simulink model "SimulacionesDT_LUCIA_con_integral"  (R2026b)
settings: Solver=ode15s  StopTime=20
values from neighbouring files (symbols this model uses):
  alpha_Cu = 3.9e-3    (= 0.0039)    [coeficientes.m]
  b_eq = b_m + b_l/(r^2)    (= 2.19444444444e-05)    [coeficientes.m]
  C_ts = 0.818    [coeficientes.m]
  g = 9.80665    [coeficientes.m]
  init_I0 = 0    [coeficientes.m]
  init_Id = 0    [coeficientes.m]
  init_Iq = 0    [coeficientes.m]
  init_theta = 0    [coeficientes.m]
  init_Ts = 20    [coeficientes.m]
  init_w = 0    [coeficientes.m]
  J_eq = J_m + J_l/(r^2)    (= 2.84652777778e-05)    [coeficientes.m]
  k_l = k_l_min + m_l*l_l    (= 0.5)    [coeficientes.m]
  Kd_mov = wn_mov * (2*zeta_mov + 1) * J_eq    (= 0.0569305555556)    [coeficientes.m]
  Ki_mov = wn_mov^3 * J_eq    (= 14574.2222222)    [coeficientes.m]
  Kp_mov = wn_mov^2 * (2*zeta_mov + 1) * J_eq    (= 45.5444444444)    [coeficientes.m]
  L_d = 6.6e-3    (= 0.0066)    [coeficientes.m]
  L_ls = 0.8e-3    (= 0.0008)    [coeficientes.m]
  L_q = 5.8e-3    (= 0.0058)    [coeficientes.m]
  lambda = 0.016    [coeficientes.m]
  Pp = 3    [coeficientes.m]
  r = 120.0    (= 120)    [coeficientes.m]
  R0 = abs(p)*L_ls    [coeficientes.m]
  R_sREF = 1.02    [coeficientes.m]
  R_tsamb = 146.7    [coeficientes.m]
  Rd = abs(p)*L_d    [coeficientes.m]
  Rq = abs(p)*L_q    [coeficientes.m]
  T_sREF = 20    [coeficientes.m]
libraries: eeTransforms x12
(part 1 of 2)
settings Model: Creator=lamun  LastModifiedBy=lamun
settings SimscapeCC: SimscapeLogType=all  SimscapeNominalValues="[{\"value\":\"1\",\"unit\":\"A\"},{\"value\":\"1\",\"unit\":\"bar\"},{\"value\":\"1\",\"unit\":\"cm^2\"},{\"value\":\"1\",\"unit\":\"cm^3/s\"},{\"value\":\"1\",\"unit\":\"kJ/kg\"},{\"value\":\"1\",\"unit\":\"kW\"},{\"value\":\"1\",\"unit\":\"l\"},{\"value\":\"1\",\"unit\":\"N\"},{\"value\":\"1\",\"unit\":\"N*m\"},{\"value\":\"1\",\"unit\":\"V\"},{\"value\":\"0.001\",\"unit\":\"Wb\"}]"  SimscapeUseEnergyAccounting=off

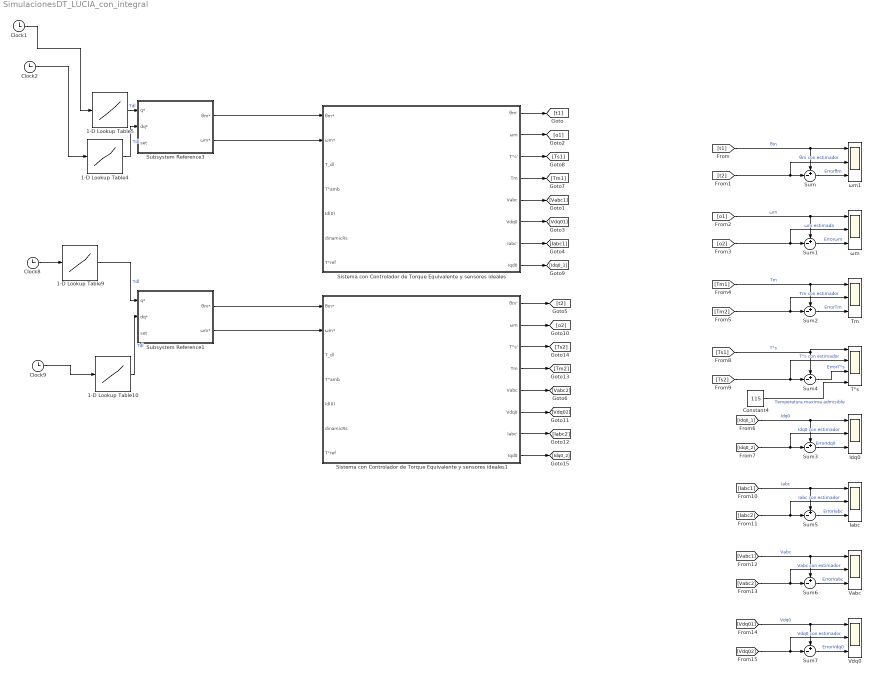
== system SimulacionesDT_LUCIA_con_integral ==
  1-D Lookup Table10 : Lookup_n-D  NumberOfTableDimensions=1  BreakpointsForDimension1=[0, 1.99, 2, 6.99, 7, 8.99, 9, 13.99, 14, 16]  Table=[0, 0, 2*pi/5, 2*pi/5, 0, 0, -2*pi/5, -2*pi/5, 0, 0]  InternalRulePriority=Speed  RndMeth=Simplest
  1-D Lookup Table4 : Lookup_n-D  NumberOfTableDimensions=1  BreakpointsForDimension1=[0, 1.99, 2, 6.99, 7, 8.99, 9, 13.99, 14, 16]  Table=[0, 0, 2*pi/5, 2*pi/5, 0, 0, -2*pi/5, -2*pi/5, 0, 0]  InternalRulePriority=Speed  RndMeth=Simplest
  1-D Lookup Table5 : Lookup_n-D  NumberOfTableDimensions=1  BreakpointsForDimension1=[0, 2, 7, 9, 14, 16]  Table=[0, 0, 2*pi, 2*pi, 0, 0]  InternalRulePriority=Speed  RndMeth=Simplest
  1-D Lookup Table9 : Lookup_n-D  NumberOfTableDimensions=1  BreakpointsForDimension1=[0, 2, 7, 9, 14, 16]  Table=[0, 0, 2*pi, 2*pi, 0, 0]  InternalRulePriority=Speed  RndMeth=Simplest
  Clock{1..2,8..9} (4 alike) : Clock
  Constant4 : Constant  Value=115
  Iabc : Scope  NumInputPorts=3
      settings: Title=Comparación Iabc  ActiveDisplayYMinimum=-616.4753395036073  ActiveDisplayYMaximum=771.0246685119215  YLabel=Iabc [A]  DataLoggingVariableName=ScopeData6
  Idq0 : Scope  NumInputPorts=3
      settings: Title=Comparación Idq0  ActiveDisplayYMinimum=-302.22808719672526  ActiveDisplayYMaximum=701.5039994194284  YLabel=Idq0 [A]  DataLoggingVariableName=ScopeData3
  Sistema con Controlador de Torque Equivalente y sensores ideales : Subsystem
  Sistema con Controlador de Torque Equivalente y sensores ideales1 : Subsystem
  Subsystem Reference1 : Subsystem
  Subsystem Reference3 : Subsystem
  Sum{,1..7} (8 alike) : Sum  Inputs=+-|
  Tm : Scope  NumInputPorts=3
      settings: Title=Comparación Torque Motor  ActiveDisplayYMinimum=-3.6327134054434631  ActiveDisplayYMaximum=3.6460056409791535  YLabel=T_m [Nm]
  T°s : Scope  NumInputPorts=4
      settings: Title=Comparación Temperatura del Estator  ActiveDisplayYMinimum=-1.4333497629401416E+11  ActiveDisplayYMaximum=1.2900147868458242E+12  YLabel=T\circ  DataLoggingVariableName=ScopeData2
  Vabc : Scope  NumInputPorts=3
      settings: Title=Comparación Vabc  ActiveDisplayYMinimum=-4.2380725007516653E+17  ActiveDisplayYMaximum=4.48793359005676E+17  YLabel=Vabc [V]  DataLoggingVariableName=ScopeData7
  Vdq0 : Scope  NumInputPorts=3
      settings: Title=Comparación Vdq0  ActiveDisplayYMinimum=-9.3011147894303968E+16  ActiveDisplayYMaximum=4.5901314557328838E+17  YLabel=Vdq0 [V]  DataLoggingVariableName=ScopeData8
  ωm : Scope  NumInputPorts=3
      settings: Title=Comparación ωm  ActiveDisplayYMinimum=-384.34516117127549  ActiveDisplayYMaximum=399.454060833598  YLabel=\omega_{motor}  DataLoggingVariableName=ScopeData5
  ωm1 : Scope  NumInputPorts=3
      settings: Title=Comparación θ motor  ActiveDisplayYMinimum=-120.08554135265514  ActiveDisplayYMaximum=869.13028937421041  YLabel=\theta_m[rad]  DataLoggingVariableName=ScopeData4
  wires:
  Sistema con Controlador de Torque Equivalente y sensores ideales1/7(Iabc') -> [Iabc2]
  [Vabc1] -> Sum6/1, Vabc/1  "Vabc"
  Sistema con Controlador de Torque Equivalente y sensores ideales1/6(Vdq0) -> [Vdq02]
  Sistema con Controlador de Torque Equivalente y sensores ideales/7(Iabc') -> [Iabc1]
  Sum1/1 -> ωm/3  "Errorωm"
  Sistema con Controlador de Torque Equivalente y sensores ideales1/8(Iqd0) -> [Idq0_2]
  Sum/1 -> ωm1/3  "Errorθm"
  Sistema con Controlador de Torque Equivalente y sensores ideales/6(Vdq0) -> [Vdq01]
  [Iabc1] -> Sum5/1, Iabc/1  "Iabc"
  Sum5/1 -> Iabc/3  "ErrorIabc"
  [Tm1] -> Tm/1, Sum2/1  "Tm"
  Subsystem Reference3/1(θm*) -> Sistema con Controlador de Torque Equivalente y sensores ideales/1(θm*)
  Sistema con Controlador de Torque Equivalente y sensores ideales/8(Iqd0) -> [Idq0_1]
  [Idq0_2] -> Idq0/2, Sum3/2  "Idq0 con estimador"
  Sum6/1 -> Vabc/3  "ErrorVabc"
  [Idq0_1] -> Sum3/1, Idq0/1  "Idq0"
  Sistema con Controlador de Torque Equivalente y sensores ideales1/3(T°s') -> [Ts2]
  [o1] -> ωm/1, Sum1/1  "ωm"
  [Vdq02] -> Vdq0/2, Sum7/2  "Vdq0 con estimador"
  Sistema con Controlador de Torque Equivalente y sensores ideales/5(Vabc) -> [Vabc1]
  Sistema con Controlador de Torque Equivalente y sensores ideales/3(T°s') -> [Ts1]
  Sistema con Controlador de Torque Equivalente y sensores ideales/1(θm') -> [t1]
  Sistema con Controlador de Torque Equivalente y sensores ideales1/2(ωm) -> [o2]
  [Tm2] -> Tm/2, Sum2/2  "Tm con estimador"
  Subsystem Reference3/2(ωm*) -> Sistema con Controlador de Torque Equivalente y sensores ideales/2(ωm*)
  Subsystem Reference1/1(θm*) -> Sistema con Controlador de Torque Equivalente y sensores ideales1/1(θm*)
  [Vdq01] -> Sum7/1, Vdq0/1  "Vdq0"
  [t2] -> ωm1/2, Sum/2  "θm con estimador"
  [t1] -> ωm1/1, Sum/1  "θm"
  Sum7/1 -> Vdq0/3  "ErrorVdq0"
  Sistema con Controlador de Torque Equivalente y sensores ideales1/4(Tm) -> [Tm2]
  Sum3/1 -> Idq0/3  "ErrorIdq0"
  Sum2/1 -> Tm/3  "ErrorTm"
  [Ts2] -> T°s/2, Sum4/2  "T°s con estimador"
  [o2] -> ωm/2, Sum1/2  "ωm estimada"
  Sum4/1 -> T°s/3  "ErrorT°s"
  Sistema con Controlador de Torque Equivalente y sensores ideales1/1(θm') -> [t2]
  Sistema con Controlador de Torque Equivalente y sensores ideales1/5(Vabc) -> [Vabc2]
  [Ts1] -> T°s/1, Sum4/1  "T°s"
  Sistema con Controlador de Torque Equivalente y sensores ideales/2(ωm) -> [o1]
  Subsystem Reference1/2(ωm*) -> Sistema con Controlador de Torque Equivalente y sensores ideales1/2(ωm*)
  [Iabc2] -> Iabc/2, Sum5/2  "Iabc con estimador"
  Sistema con Controlador de Torque Equivalente y sensores ideales/4(Tm) -> [Tm1]
  [Vabc2] -> Vabc/2, Sum6/2  "Vabc con estimador"
  Constant4/1 -> T°s/4  "Temperatura maxima admisible"
  Clock2/1 -> 1-D Lookup Table4/1
  Clock1/1 -> 1-D Lookup Table5/1
  Clock9/1 -> 1-D Lookup Table10/1
  Clock8/1 -> 1-D Lookup Table9/1
  1-D Lookup Table9/1 -> Subsystem Reference1/1(q*)  "Tdl"
  1-D Lookup Table10/1 -> Subsystem Reference1/2(dq*)  "Tdl"
  1-D Lookup Table4/1 -> Subsystem Reference3/2(dq*)  "Tdl"
  1-D Lookup Table5/1 -> Subsystem Reference3/1(q*)  "Tdl"

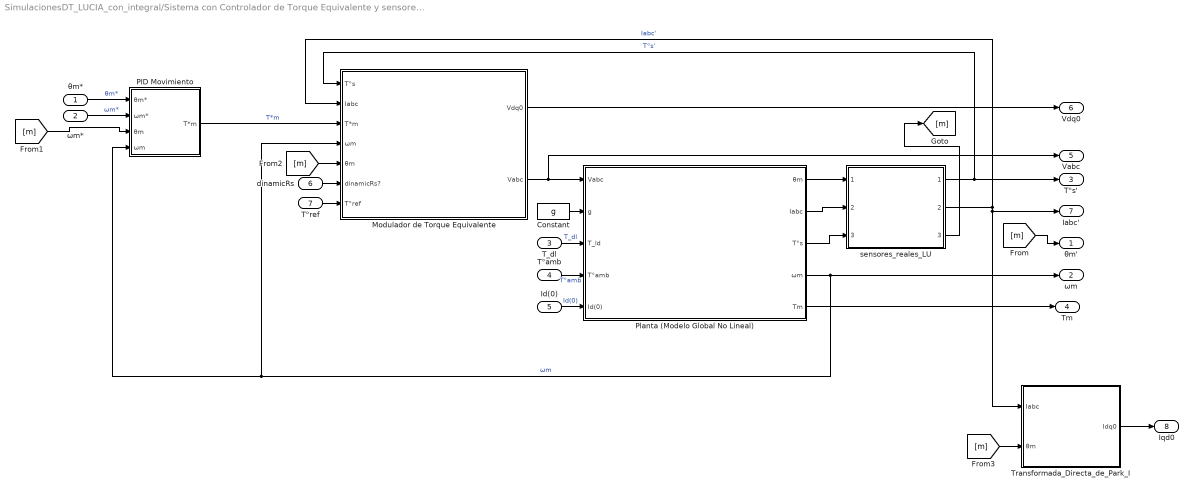
== system SimulacionesDT_LUCIA_con_integral/Sistema con Controlador de Torque Equivalente y sensores ideales ==
  θm* : Inport
  ωm* : Inport  Port=2
  T_dl : Inport  Port=3
  T°amb : Inport  Port=4
  Id(0) : Inport  Port=5
  dinamicRs : Inport  Port=6
  T°ref : Inport  Port=7
  Constant : Constant  Value=g
  Modulador de Torque Equivalente : Subsystem
      settings: PortSchema="{\"entries\":[{\"content\":{\"sides\":[{\"content\":{\"connectorIds\":[\"In1\",\"In3\",\"In5\",\"In2\",\"In4\",\"In6\",\"In7\"]},\"type\":\"ConnectorPlacement.EquallySpacedRectSide\",\"uuid\":\"ea9ad4ab-f607-4d37-9442-85f6cfda2486\"},{\"content\":{\"connectorIds\":[\"Out2\",\"Out1\"],\"side\":\"RIGHT\"},\"type\":\"ConnectorPlacement.EquallySpacedRectSide\",\"uuid\":\"696b5fe5-1f6c-4fc9-932e-86b56d49996f\"},{\"content\":{\"side\":\"TOP\"},\"type\":\"ConnectorPlacement.EquallySpacedRectSide\",\"uuid\":\"45e3ac4c-5a2f-4a79-9454-e497b07295c7\"}]},\"type\":\"ConnectorPlacement.EquallySpacedConnector\",\"uuid\":\"ad401c21-3c60-4ab4-96eb-f449fc93609a\"}],\"packageUris\":[\"http://schema.mathworks.com/mf0/Connector/R2020b\"],\"version\":\"1.0\"}"
  PID Movimiento : Subsystem
      settings: PortSchema="{\"entries\":[{\"content\":{\"sides\":[{\"content\":{\"connectorIds\":[\"In3\",\"In4\",\"In2\",\"In1\"]},\"type\":\"ConnectorPlacement.EquallySpacedRectSide\",\"uuid\":\"99b9ec4b-f651-40ed-8a16-085c2c4ac88d\"},{\"content\":{\"connectorIds\":[\"Out1\"],\"side\":\"RIGHT\"},\"type\":\"ConnectorPlacement.EquallySpacedRectSide\",\"uuid\":\"009a9369-fd86-4ac2-a423-7c7f1491457b\"},{\"content\":{\"side\":\"TOP\"},\"type\":\"ConnectorPlacement.EquallySpacedRectSide\",\"uuid\":\"0bc889a5-9100-482e-a11a-4c36993d76f7\"}]},\"type\":\"ConnectorPlacement.EquallySpacedConnector\",\"uuid\":\"de270b8a-8a15-46e7-87f3-10db7988a399\"}],\"packageUris\":[\"http://schema.mathworks.com/mf0/Connector/R2020b\"],\"version\":\"1.0\"}"
  Planta (Modelo Global No Lineal) : Subsystem
      settings: PortSchema="{\"entries\":[{\"content\":{\"sides\":[{\"content\":{\"connectorIds\":[\"In1\",\"In3\",\"In2\",\"In4\",\"In5\"]},\"type\":\"ConnectorPlacement.EquallySpacedRectSide\",\"uuid\":\"3481abf0-b0cb-49f6-b93f-5a31fbfa4119\"},{\"content\":{\"connectorIds\":[\"Out1\",\"Out2\",\"Out3\",\"Out4\",\"Out5\"],\"side\":\"RIGHT\"},\"type\":\"ConnectorPlacement.EquallySpacedRectSide\",\"uuid\":\"81dbc61e-d5f3-4edc-bc73-ec3d6160a008\"},{\"content\":{\"side\":\"TOP\"},\"type\":\"ConnectorPlacement.EquallySpacedRectSide\",\"uuid\":\"48e37594-92fb-4835-b4aa-9211b8b6a309\"}]},\"type\":\"ConnectorPlacement.EquallySpacedConnector\",\"uuid\":\"6c32b8e1-5803-41f4-af4e-ba3a494349ba\"}],\"packageUris\":[\"http://schema.mathworks.com/mf0/Connector/R2020b\"],\"version\":\"1.0\"}"
  Transformada_Directa_de_Park_I : Subsystem
  sensores_reales_LU : Subsystem  ReferencedSubsystem=sensores_reales_LU
  θm' : Outport
  ωm : Outport  Port=2
  T°s' : Outport  Port=3
  Tm : Outport  Port=4
  Vabc : Outport  Port=5  OutDataTypeStr=Bus: Vabc
  Vdq0 : Outport  Port=6  OutDataTypeStr=Bus: Vdq0
  Iabc' : Outport  Port=7  OutDataTypeStr=Bus: Iabc
  Iqd0 : Outport  Port=8  OutDataTypeStr=Bus: Idq0
  wires:
  Transformada_Directa_de_Park_I/1(Idq0) -> Iqd0/1
  T°ref/1 -> Modulador de Torque Equivalente/7(T°ref)
  dinamicRs/1 -> Modulador de Torque Equivalente/6(dinamicRs?)
  Modulador de Torque Equivalente/2(Vdq0) -> Vdq0/1
  Planta (Modelo Global No Lineal)/5(Tm) -> Tm/1
  T_dl/1 -> Planta (Modelo Global No Lineal)/2(T_ld)  "T_dl"
  T°amb/1 -> Planta (Modelo Global No Lineal)/4(T°amb)  "T°amb"
  Id(0)/1 -> Planta (Modelo Global No Lineal)/5(Id(0))  "Id(0)"
  Constant/1 -> Planta (Modelo Global No Lineal)/3(g)
  sensores_reales_LU/1 -> T°s'/1, Modulador de Torque Equivalente/1(T°s)  "T°s'"
  sensores_reales_LU/2 -> Transformada_Directa_de_Park_I/1(Iabc), Iabc'/1, Modulador de Torque Equivalente/3(Iabc)  "Iabc'"
  Planta (Modelo Global No Lineal)/3(T°s) -> sensores_reales_LU/3
  Modulador de Torque Equivalente/1(Vabc) -> Vabc/1, Planta (Modelo Global No Lineal)/1(Vabc)
  Planta (Modelo Global No Lineal)/2(Iabc) -> sensores_reales_LU/2
  Planta (Modelo Global No Lineal)/1(θm) -> sensores_reales_LU/1
  θm*/1 -> PID Movimiento/3(θm*)  "θm*"
  PID Movimiento/1(T*m) -> Modulador de Torque Equivalente/5(T*m)  "T*m"
  ωm*/1 -> PID Movimiento/4(ωm*)  "ωm*"
  Planta (Modelo Global No Lineal)/4(ωm) -> PID Movimiento/1(ωm), Modulador de Torque Equivalente/2(ωm), ωm/1  "ωm"
  sensores_reales_LU/3 -> [m]
  [m] -> θm'/1
  [m] -> PID Movimiento/2(θm)
  [m] -> Modulador de Torque Equivalente/4(θm)
  [m] -> Transformada_Directa_de_Park_I/2(θm)

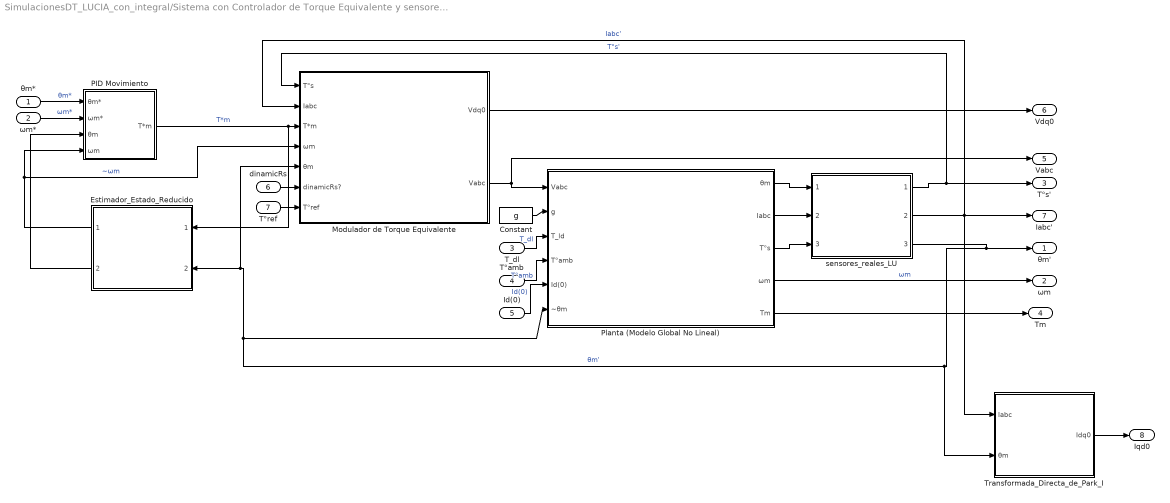
== system SimulacionesDT_LUCIA_con_integral/Sistema con Controlador de Torque Equivalente y sensores ideales1 ==
  θm* : Inport
  ωm* : Inport  Port=2
  T_dl : Inport  Port=3
  T°amb : Inport  Port=4
  Id(0) : Inport  Port=5
  dinamicRs : Inport  Port=6
  T°ref : Inport  Port=7
  Constant : Constant  Value=g
  Estimador_Estado_Reducido : Subsystem  ReferencedSubsystem=Estimador_Estado_Reducido
  Modulador de Torque Equivalente : Subsystem
      settings: PortSchema="{\"entries\":[{\"content\":{\"sides\":[{\"content\":{\"connectorIds\":[\"In1\",\"In3\",\"In5\",\"In2\",\"In4\",\"In6\",\"In7\"]},\"type\":\"ConnectorPlacement.EquallySpacedRectSide\",\"uuid\":\"ea9ad4ab-f607-4d37-9442-85f6cfda2486\"},{\"content\":{\"connectorIds\":[\"Out2\",\"Out1\"],\"side\":\"RIGHT\"},\"type\":\"ConnectorPlacement.EquallySpacedRectSide\",\"uuid\":\"696b5fe5-1f6c-4fc9-932e-86b56d49996f\"},{\"content\":{\"side\":\"TOP\"},\"type\":\"ConnectorPlacement.EquallySpacedRectSide\",\"uuid\":\"45e3ac4c-5a2f-4a79-9454-e497b07295c7\"}]},\"type\":\"ConnectorPlacement.EquallySpacedConnector\",\"uuid\":\"ad401c21-3c60-4ab4-96eb-f449fc93609a\"}],\"packageUris\":[\"http://schema.mathworks.com/mf0/Connector/R2020b\"],\"version\":\"1.0\"}"
  PID Movimiento : Subsystem
      settings: PortSchema="{\"entries\":[{\"content\":{\"sides\":[{\"content\":{\"connectorIds\":[\"In3\",\"In4\",\"In2\",\"In1\"]},\"type\":\"ConnectorPlacement.EquallySpacedRectSide\",\"uuid\":\"99b9ec4b-f651-40ed-8a16-085c2c4ac88d\"},{\"content\":{\"connectorIds\":[\"Out1\"],\"side\":\"RIGHT\"},\"type\":\"ConnectorPlacement.EquallySpacedRectSide\",\"uuid\":\"009a9369-fd86-4ac2-a423-7c7f1491457b\"},{\"content\":{\"side\":\"TOP\"},\"type\":\"ConnectorPlacement.EquallySpacedRectSide\",\"uuid\":\"0bc889a5-9100-482e-a11a-4c36993d76f7\"}]},\"type\":\"ConnectorPlacement.EquallySpacedConnector\",\"uuid\":\"de270b8a-8a15-46e7-87f3-10db7988a399\"}],\"packageUris\":[\"http://schema.mathworks.com/mf0/Connector/R2020b\"],\"version\":\"1.0\"}"
  Planta (Modelo Global No Lineal) : Subsystem
      settings: PortSchema="{\"entries\":[{\"content\":{\"sides\":[{\"content\":{\"connectorIds\":[\"In1\",\"In3\",\"In2\",\"In4\",\"In5\",\"In6\"]},\"type\":\"ConnectorPlacement.EquallySpacedRectSide\",\"uuid\":\"3481abf0-b0cb-49f6-b93f-5a31fbfa4119\"},{\"content\":{\"connectorIds\":[\"Out1\",\"Out2\",\"Out3\",\"Out4\",\"Out5\"],\"side\":\"RIGHT\"},\"type\":\"ConnectorPlacement.EquallySpacedRectSide\",\"uuid\":\"81dbc61e-d5f3-4edc-bc73-ec3d6160a008\"},{\"content\":{\"side\":\"TOP\"},\"type\":\"ConnectorPlacement.EquallySpacedRectSide\",\"uuid\":\"48e37594-92fb-4835-b4aa-9211b8b6a309\"}]},\"type\":\"ConnectorPlacement.EquallySpacedConnector\",\"uuid\":\"6c32b8e1-5803-41f4-af4e-ba3a494349ba\"}],\"packageUris\":[\"http://schema.mathworks.com/mf0/Connector/R2020b\"],\"version\":\"1.0\"}"
  Transformada_Directa_de_Park_I : Subsystem
  sensores_reales_LU : Subsystem  ReferencedSubsystem=sensores_reales_LU
  θm' : Outport
  ωm : Outport  Port=2
  T°s' : Outport  Port=3
  Tm : Outport  Port=4
  Vabc : Outport  Port=5  OutDataTypeStr=Bus: Vabc
  Vdq0 : Outport  Port=6  OutDataTypeStr=Bus: Vdq0
  Iabc' : Outport  Port=7  OutDataTypeStr=Bus: Iabc
  Iqd0 : Outport  Port=8  OutDataTypeStr=Bus: Idq0
  wires:
  Transformada_Directa_de_Park_I/1(Idq0) -> Iqd0/1
  T°ref/1 -> Modulador de Torque Equivalente/7(T°ref)
  dinamicRs/1 -> Modulador de Torque Equivalente/6(dinamicRs?)
  Modulador de Torque Equivalente/2(Vdq0) -> Vdq0/1
  Planta (Modelo Global No Lineal)/5(Tm) -> Tm/1
  T_dl/1 -> Planta (Modelo Global No Lineal)/2(T_ld)  "T_dl"
  T°amb/1 -> Planta (Modelo Global No Lineal)/4(T°amb)  "T°amb"
  Id(0)/1 -> Planta (Modelo Global No Lineal)/5(Id(0))  "Id(0)"
  Constant/1 -> Planta (Modelo Global No Lineal)/3(g)
  sensores_reales_LU/1 -> Modulador de Torque Equivalente/1(T°s), T°s'/1  "T°s'"
  sensores_reales_LU/2 -> Transformada_Directa_de_Park_I/1(Iabc), Iabc'/1, Modulador de Torque Equivalente/3(Iabc)  "Iabc'"
  Planta (Modelo Global No Lineal)/3(T°s) -> sensores_reales_LU/3
  Modulador de Torque Equivalente/1(Vabc) -> Vabc/1, Planta (Modelo Global No Lineal)/1(Vabc)
  Planta (Modelo Global No Lineal)/2(Iabc) -> sensores_reales_LU/2
  sensores_reales_LU/3 -> Estimador_Estado_Reducido/2, Modulador de Torque Equivalente/4(θm), Planta (Modelo Global No Lineal)/6(~θm), Transformada_Directa_de_Park_I/2(θm), θm'/1  "θm'"
  Planta (Modelo Global No Lineal)/1(θm) -> sensores_reales_LU/1
  θm*/1 -> PID Movimiento/3(θm*)  "θm*"
  PID Movimiento/1(T*m) -> Estimador_Estado_Reducido/1, Modulador de Torque Equivalente/5(T*m)  "T*m"
  Estimador_Estado_Reducido/1 -> PID Movimiento/1(ωm), Modulador de Torque Equivalente/2(ωm)  "~ωm"
  ωm*/1 -> PID Movimiento/4(ωm*)  "ωm*"
  Planta (Modelo Global No Lineal)/4(ωm) -> ωm/1  "ωm"
  Estimador_Estado_Reducido/2 -> PID Movimiento/2(θm)

== system SimulacionesDT_LUCIA_con_integral/Subsystem Reference1 ==
  q* : Inport
  dq* : Inport  Port=2
  set : Inport  Port=3
  Gain : Gain  Gain=r
  Gain1 : Gain  Gain=r
  Integrator : Integrator  ExternalReset=level  InitialConditionSource=external
  Selector : RelationalOperator  Operator=>  OutDataTypeStr=boolean  RndMeth=Simplest  InputSameDT=off
  Switch : Switch  Criteria=u2 ~= 0  SaturateOnIntegerOverflow=off  InputSameDT=off
  Umbral : Constant  Value=0.5
  θm* : Outport
  ωm* : Outport  Port=2
  wires:
  Switch/1 -> θm*/1
  Integrator/1 -> Switch/3
  Gain1/1 -> ωm*/1, Integrator/1
  Selector/1 -> Switch/2, Integrator/2
  Gain/1 -> Switch/1, Integrator/3
  Umbral/1 -> Selector/2
  set/1 -> Selector/1
  dq*/1 -> Gain1/1
  q*/1 -> Gain/1

== system SimulacionesDT_LUCIA_con_integral/Subsystem Reference3 ==
  q* : Inport
  dq* : Inport  Port=2
  set : Inport  Port=3
  Gain : Gain  Gain=r
  Gain1 : Gain  Gain=r
  Integrator : Integrator  ExternalReset=level  InitialConditionSource=external
  Selector : RelationalOperator  Operator=>  OutDataTypeStr=boolean  RndMeth=Simplest  InputSameDT=off
  Switch : Switch  Criteria=u2 ~= 0  SaturateOnIntegerOverflow=off  InputSameDT=off
  Umbral : Constant  Value=0.5
  θm* : Outport
  ωm* : Outport  Port=2
  wires:
  q*/1 -> Gain/1
  dq*/1 -> Gain1/1
  set/1 -> Selector/1
  Umbral/1 -> Selector/2
  Gain/1 -> Integrator/3, Switch/1
  Selector/1 -> Integrator/2, Switch/2
  Gain1/1 -> Integrator/1, ωm*/1
  Integrator/1 -> Switch/3
  Switch/1 -> θm*/1

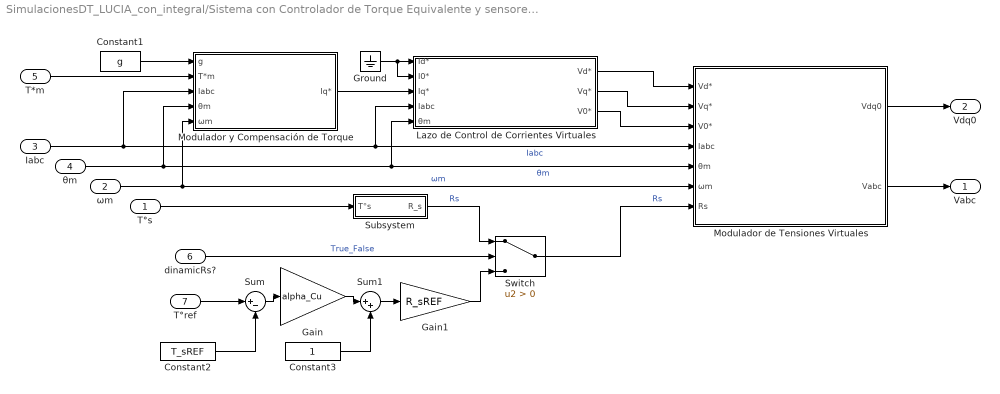
== system SimulacionesDT_LUCIA_con_integral/Sistema con Controlador de Torque Equivalente y sensores ideales/Modulador de Torque Equivalente ==
  T°s : Inport
  ωm : Inport  Port=2
  Iabc : Inport  Port=3
  θm : Inport  Port=4
  T*m : Inport  Port=5
  dinamicRs? : Inport  Port=6
  T°ref : Inport  Port=7
  Constant1 : Constant  Value=g
  Constant2 : Constant  Value=T_sREF
  Constant3 : Constant
  Gain : Gain  Gain=alpha_Cu
  Gain1 : Gain  Gain=R_sREF
  Ground : Ground
  Lazo de Control de Corrientes Virtuales : Subsystem
      settings: PortSchema="{\"entries\":[{\"content\":{\"sides\":[{\"content\":{\"connectorIds\":[\"In2\",\"In3\",\"In1\",\"In4\",\"In5\"]},\"type\":\"ConnectorPlacement.EquallySpacedRectSide\",\"uuid\":\"7378df2b-1b9c-42cd-9ef6-9bfa4de31228\"},{\"content\":{\"connectorIds\":[\"Out2\",\"Out1\",\"Out3\"],\"side\":\"RIGHT\"},\"type\":\"ConnectorPlacement.EquallySpacedRectSide\",\"uuid\":\"75ac4e09-b611-4ee2-aa1e-16791f3f98b8\"},{\"content\":{\"side\":\"TOP\"},\"type\":\"ConnectorPlacement.EquallySpacedRectSide\",\"uuid\":\"c32b7829-5b6a-417b-8aae-eaa4caf59bef\"}]},\"type\":\"ConnectorPlacement.EquallySpacedConnector\",\"uuid\":\"1d84f5ff-db01-492a-bfe1-22065b3eebb0\"}],\"packageUris\":[\"http://schema.mathworks.com/mf0/Connector/R2020b\"],\"version\":\"1.0\"}"
  Modulador de Tensiones Virtuales : Subsystem
      settings: PortSchema="{\"entries\":[{\"content\":{\"sides\":[{\"content\":{\"connectorIds\":[\"In2\",\"In1\",\"In3\",\"In6\",\"In7\",\"In5\",\"In4\"]},\"type\":\"ConnectorPlacement.EquallySpacedRectSide\",\"uuid\":\"561a625a-719f-47d4-85d3-a88e423068dd\"},{\"content\":{\"connectorIds\":[\"Out2\",\"Out1\"],\"side\":\"RIGHT\"},\"type\":\"ConnectorPlacement.EquallySpacedRectSide\",\"uuid\":\"c1cdd74a-6c1d-470e-a6ac-8d72e83b5cc5\"},{\"content\":{\"side\":\"TOP\"},\"type\":\"ConnectorPlacement.EquallySpacedRectSide\",\"uuid\":\"c5935c6f-534c-46b9-aa64-6d6dabbbb210\"}]},\"type\":\"ConnectorPlacement.EquallySpacedConnector\",\"uuid\":\"b0debde9-6e18-4e06-b0c4-28c9c51e472d\"}],\"packageUris\":[\"http://schema.mathworks.com/mf0/Connector/R2020b\"],\"version\":\"1.0\"}"
  Modulador y Compensación de Torque : Subsystem
      settings: PortSchema="{\"entries\":[{\"content\":{\"sides\":[{\"content\":{\"connectorIds\":[\"In5\",\"In1\",\"In2\",\"In3\",\"In4\"]},\"type\":\"ConnectorPlacement.EquallySpacedRectSide\",\"uuid\":\"ea9ad4ab-f607-4d37-9442-85f6cfda2486\"},{\"content\":{\"connectorIds\":[\"Out1\"],\"side\":\"RIGHT\"},\"type\":\"ConnectorPlacement.EquallySpacedRectSide\",\"uuid\":\"696b5fe5-1f6c-4fc9-932e-86b56d49996f\"},{\"content\":{\"side\":\"TOP\"},\"type\":\"ConnectorPlacement.EquallySpacedRectSide\",\"uuid\":\"45e3ac4c-5a2f-4a79-9454-e497b07295c7\"}]},\"type\":\"ConnectorPlacement.EquallySpacedConnector\",\"uuid\":\"ad401c21-3c60-4ab4-96eb-f449fc93609a\"}],\"packageUris\":[\"http://schema.mathworks.com/mf0/Connector/R2020b\"],\"version\":\"1.0\"}"
  Subsystem : Subsystem
  Sum : Sum  Inputs=|+-
  Sum1 : Sum  Inputs=|++
  Switch : Switch  Criteria=u2 > Threshold  SaturateOnIntegerOverflow=off  InputSameDT=off
  Vabc : Outport
  Vdq0 : Outport  Port=2
  wires:
  Sum1/1 -> Gain1/1
  Constant3/1 -> Sum1/2
  Gain/1 -> Sum1/1
  Sum/1 -> Gain/1
  Constant2/1 -> Sum/2
  T°ref/1 -> Sum/1
  Constant1/1 -> Modulador y Compensación de Torque/5(g)
  Modulador de Tensiones Virtuales/2(Vdq0) -> Vdq0/1
  Gain1/1 -> Switch/3
  Switch/1 -> Modulador de Tensiones Virtuales/4(Rs)  "Rs"
  dinamicRs?/1 -> Switch/2  "True_False"
  Subsystem/1(R_s) -> Switch/1  "Rs"
  T°s/1 -> Subsystem/1(T°s)
  Iabc/1 -> Modulador y Compensación de Torque/2(Iabc), Lazo de Control de Corrientes Virtuales/4(Iabc), Modulador de Tensiones Virtuales/6(Iabc)  "Iabc"
  Ground/1 -> Lazo de Control de Corrientes Virtuales/3(I0*), Lazo de Control de Corrientes Virtuales/2(Id*)
  Modulador de Tensiones Virtuales/1(Vabc) -> Vabc/1
  ωm/1 -> Modulador y Compensación de Torque/4(ωm), Modulador de Tensiones Virtuales/5(ωm)  "ωm"
  θm/1 -> Modulador y Compensación de Torque/3(θm), Lazo de Control de Corrientes Virtuales/5(θm), Modulador de Tensiones Virtuales/7(θm)  "θm"
  T*m/1 -> Modulador y Compensación de Torque/1(T*m)
  Modulador y Compensación de Torque/1(Iq*) -> Lazo de Control de Corrientes Virtuales/1(Iq*)
  Lazo de Control de Corrientes Virtuales/3(V0*) -> Modulador de Tensiones Virtuales/3(V0*)
  Lazo de Control de Corrientes Virtuales/2(Vd*) -> Modulador de Tensiones Virtuales/2(Vd*)
  Lazo de Control de Corrientes Virtuales/1(Vq*) -> Modulador de Tensiones Virtuales/1(Vq*)

== system SimulacionesDT_LUCIA_con_integral/Sistema con Controlador de Torque Equivalente y sensores ideales/PID Movimiento ==
  ωm : Inport  Unit=rad/s
  θm : Inport  Port=2
  θm* : Inport  Port=3  Unit=rad/s
  ωm* : Inport  Port=4  Unit=rad/s
  Gain : Gain  Gain=Kd_mov
  Gain1 : Gain  Gain=Kp_mov
  Gain2 : Gain  Gain=Ki_mov
  Integrator1 : Integrator
  Sum : Sum  Inputs=|+-
  Sum1 : Sum  Inputs=+++
  Sum2 : Sum  Inputs=|+-
  T*m : Outport
  wires:
  Gain1/1 -> Sum1/2
  Sum1/1 -> T*m/1
  Gain2/1 -> Sum1/1
  Gain/1 -> Sum1/3
  θm*/1 -> Sum2/1
  Sum/1 -> Gain/1  "eω"
  θm/1 -> Sum2/2
  ωm*/1 -> Sum/1
  ωm/1 -> Sum/2
  Integrator1/1 -> Gain2/1  "e∫θ"
  Sum2/1 -> Gain1/1, Integrator1/1  "eθ"

== system SimulacionesDT_LUCIA_con_integral/Sistema con Controlador de Torque Equivalente y sensores ideales/Planta (Modelo Global No Lineal) ==
  note: Sistema Global No Lineal
  Vabc : Inport  OutDataTypeStr=Bus: Vabc
  T_ld : Inport  Port=2
  g : Inport  Port=3
  T°amb : Inport  Port=4
  Id(0) : Inport  Port=5
  Bus Selector : BusSelector  OutputSignals=Vd,Vq,V0
  Gain : Gain  Gain=Pp
  Subsistema Electromagnetico : Subsystem
  Subsistema Mecanico Equivalente : Subsystem
  Subsistema Termico : Subsystem
  Transformada Directa de Park : Subsystem
  Transformada Inversa de Park : Subsystem  ReferencedSubsystem=Transformada_Inversa_de_Park_I
  θm : Outport
  Iabc : Outport  Port=2  OutDataTypeStr=Bus: Iabc
  T°s : Outport  Port=3
  ωm : Outport  Port=4
  Tm : Outport  Port=5
  wires:
  Id(0)/1 -> Subsistema Electromagnetico/6(Id(0))
  Transformada Inversa de Park/1 -> Iabc/1  "Iabc"
  Bus Selector/3 -> Subsistema Electromagnetico/5(V0)  "<V0>"
  Bus Selector/2 -> Subsistema Electromagnetico/4(Vq)  "<Vq>"
  Bus Selector/1 -> Subsistema Electromagnetico/3(Vd)  "<Vd>"
  Transformada Directa de Park/1(Vdq0) -> Bus Selector/1
  g/1 -> Subsistema Mecanico Equivalente/3(g)
  T°amb/1 -> Subsistema Termico/2(T°amb)
  Vabc/1 -> Transformada Directa de Park/1(Vabc)
  T_ld/1 -> Subsistema Mecanico Equivalente/2(T_ld)
  Gain/1 -> Subsistema Electromagnetico/2(ωr)
  Subsistema Termico/1(R_s) -> Subsistema Electromagnetico/1(R_s)
  Subsistema Electromagnetico/2(T_m) -> Tm/1, Subsistema Mecanico Equivalente/1(T_m)  "Tm"
  Subsistema Mecanico Equivalente/2(θm) -> θm/1, Transformada Inversa de Park/2, Transformada Directa de Park/2(θm)  "θm"
  Subsistema Mecanico Equivalente/1(ωm) -> ωm/1, Gain/1  "ωm"
  Subsistema Electromagnetico/1(Idq0) -> Transformada Inversa de Park/1, Subsistema Termico/1(Idq0)  "Idq0"
  Subsistema Termico/2(T°s) -> T°s/1  "T°s"

== system SimulacionesDT_LUCIA_con_integral/Sistema con Controlador de Torque Equivalente y sensores ideales/Transformada_Directa_de_Park_I ==
  Iabc : Inport  OutDataTypeStr=Bus: Iabc
  θm : Inport  Port=2
  Ancho_abc : SignalSpecification  Dimensions=3
  Bus Creator : BusCreator  Inputs=3
  Bus to Vector : BusToVector
  Demux : Demux  Outputs=3
  Gain3 : Gain  Gain=Pp
  Park Transform : eeTransforms/Park Transform  AxisAlignment=Q-axis  PowerInvariant=off
      settings: LibrarySourceBlock=|
      | ee_sl_lib/Mathematical
      | Transforms/Park Transform
  Idq0 : Outport  OutDataTypeStr=Bus: Idq0
  wires:
  Ancho_abc/1 -> Park Transform/1
  Bus to Vector/1 -> Ancho_abc/1
  θm/1 -> Gain3/1
  Iabc/1 -> Bus to Vector/1
  Bus Creator/1 -> Idq0/1
  Demux/2 -> Bus Creator/2  "Iq"
  Demux/3 -> Bus Creator/3  "I0"
  Demux/1 -> Bus Creator/1  "Id"
  Park Transform/1 -> Demux/1  "Idq0"
  Gain3/1 -> Park Transform/2

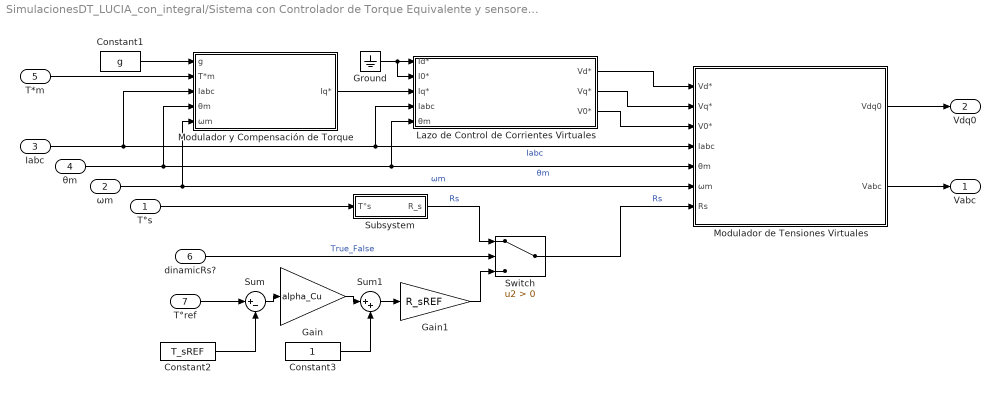
== system SimulacionesDT_LUCIA_con_integral/Sistema con Controlador de Torque Equivalente y sensores ideales1/Modulador de Torque Equivalente ==
  T°s : Inport
  ωm : Inport  Port=2
  Iabc : Inport  Port=3
  θm : Inport  Port=4
  T*m : Inport  Port=5
  dinamicRs? : Inport  Port=6
  T°ref : Inport  Port=7
  Constant1 : Constant  Value=g
  Constant2 : Constant  Value=T_sREF
  Constant3 : Constant
  Gain : Gain  Gain=alpha_Cu
  Gain1 : Gain  Gain=R_sREF
  Ground : Ground
  Lazo de Control de Corrientes Virtuales : Subsystem
      settings: PortSchema="{\"entries\":[{\"content\":{\"sides\":[{\"content\":{\"connectorIds\":[\"In2\",\"In3\",\"In1\",\"In4\",\"In5\"]},\"type\":\"ConnectorPlacement.EquallySpacedRectSide\",\"uuid\":\"7378df2b-1b9c-42cd-9ef6-9bfa4de31228\"},{\"content\":{\"connectorIds\":[\"Out2\",\"Out1\",\"Out3\"],\"side\":\"RIGHT\"},\"type\":\"ConnectorPlacement.EquallySpacedRectSide\",\"uuid\":\"75ac4e09-b611-4ee2-aa1e-16791f3f98b8\"},{\"content\":{\"side\":\"TOP\"},\"type\":\"ConnectorPlacement.EquallySpacedRectSide\",\"uuid\":\"c32b7829-5b6a-417b-8aae-eaa4caf59bef\"}]},\"type\":\"ConnectorPlacement.EquallySpacedConnector\",\"uuid\":\"1d84f5ff-db01-492a-bfe1-22065b3eebb0\"}],\"packageUris\":[\"http://schema.mathworks.com/mf0/Connector/R2020b\"],\"version\":\"1.0\"}"
  Modulador de Tensiones Virtuales : Subsystem
      settings: PortSchema="{\"entries\":[{\"content\":{\"sides\":[{\"content\":{\"connectorIds\":[\"In2\",\"In1\",\"In3\",\"In6\",\"In7\",\"In5\",\"In4\"]},\"type\":\"ConnectorPlacement.EquallySpacedRectSide\",\"uuid\":\"561a625a-719f-47d4-85d3-a88e423068dd\"},{\"content\":{\"connectorIds\":[\"Out2\",\"Out1\"],\"side\":\"RIGHT\"},\"type\":\"ConnectorPlacement.EquallySpacedRectSide\",\"uuid\":\"c1cdd74a-6c1d-470e-a6ac-8d72e83b5cc5\"},{\"content\":{\"side\":\"TOP\"},\"type\":\"ConnectorPlacement.EquallySpacedRectSide\",\"uuid\":\"c5935c6f-534c-46b9-aa64-6d6dabbbb210\"}]},\"type\":\"ConnectorPlacement.EquallySpacedConnector\",\"uuid\":\"b0debde9-6e18-4e06-b0c4-28c9c51e472d\"}],\"packageUris\":[\"http://schema.mathworks.com/mf0/Connector/R2020b\"],\"version\":\"1.0\"}"
  Modulador y Compensación de Torque : Subsystem
      settings: PortSchema="{\"entries\":[{\"content\":{\"sides\":[{\"content\":{\"connectorIds\":[\"In5\",\"In1\",\"In2\",\"In3\",\"In4\"]},\"type\":\"ConnectorPlacement.EquallySpacedRectSide\",\"uuid\":\"ea9ad4ab-f607-4d37-9442-85f6cfda2486\"},{\"content\":{\"connectorIds\":[\"Out1\"],\"side\":\"RIGHT\"},\"type\":\"ConnectorPlacement.EquallySpacedRectSide\",\"uuid\":\"696b5fe5-1f6c-4fc9-932e-86b56d49996f\"},{\"content\":{\"side\":\"TOP\"},\"type\":\"ConnectorPlacement.EquallySpacedRectSide\",\"uuid\":\"45e3ac4c-5a2f-4a79-9454-e497b07295c7\"}]},\"type\":\"ConnectorPlacement.EquallySpacedConnector\",\"uuid\":\"ad401c21-3c60-4ab4-96eb-f449fc93609a\"}],\"packageUris\":[\"http://schema.mathworks.com/mf0/Connector/R2020b\"],\"version\":\"1.0\"}"
  Subsystem : Subsystem
  Sum : Sum  Inputs=|+-
  Sum1 : Sum  Inputs=|++
  Switch : Switch  Criteria=u2 > Threshold  SaturateOnIntegerOverflow=off  InputSameDT=off
  Vabc : Outport
  Vdq0 : Outport  Port=2
  wires:
  Sum1/1 -> Gain1/1
  Constant3/1 -> Sum1/2
  Gain/1 -> Sum1/1
  Sum/1 -> Gain/1
  Constant2/1 -> Sum/2
  T°ref/1 -> Sum/1
  Constant1/1 -> Modulador y Compensación de Torque/5(g)
  Modulador de Tensiones Virtuales/2(Vdq0) -> Vdq0/1
  Gain1/1 -> Switch/3
  Switch/1 -> Modulador de Tensiones Virtuales/4(Rs)  "Rs"
  dinamicRs?/1 -> Switch/2  "True_False"
  Subsystem/1(R_s) -> Switch/1  "Rs"
  T°s/1 -> Subsystem/1(T°s)
  Iabc/1 -> Modulador y Compensación de Torque/2(Iabc), Lazo de Control de Corrientes Virtuales/4(Iabc), Modulador de Tensiones Virtuales/6(Iabc)  "Iabc"
  Ground/1 -> Lazo de Control de Corrientes Virtuales/3(I0*), Lazo de Control de Corrientes Virtuales/2(Id*)
  Modulador de Tensiones Virtuales/1(Vabc) -> Vabc/1
  ωm/1 -> Modulador y Compensación de Torque/4(ωm), Modulador de Tensiones Virtuales/5(ωm)  "ωm"
  θm/1 -> Modulador y Compensación de Torque/3(θm), Lazo de Control de Corrientes Virtuales/5(θm), Modulador de Tensiones Virtuales/7(θm)  "θm"
  T*m/1 -> Modulador y Compensación de Torque/1(T*m)
  Modulador y Compensación de Torque/1(Iq*) -> Lazo de Control de Corrientes Virtuales/1(Iq*)
  Lazo de Control de Corrientes Virtuales/3(V0*) -> Modulador de Tensiones Virtuales/3(V0*)
  Lazo de Control de Corrientes Virtuales/2(Vd*) -> Modulador de Tensiones Virtuales/2(Vd*)
  Lazo de Control de Corrientes Virtuales/1(Vq*) -> Modulador de Tensiones Virtuales/1(Vq*)

== system SimulacionesDT_LUCIA_con_integral/Sistema con Controlador de Torque Equivalente y sensores ideales1/PID Movimiento ==
  ωm : Inport  Unit=rad/s
  θm : Inport  Port=2
  θm* : Inport  Port=3  Unit=rad/s
  ωm* : Inport  Port=4  Unit=rad/s
  Gain : Gain  Gain=Kd_mov
  Gain1 : Gain  Gain=Kp_mov
  Gain2 : Gain  Gain=Ki_mov
  Integrator1 : Integrator
  Sum : Sum  Inputs=|+-
  Sum1 : Sum  Inputs=+++
  Sum2 : Sum  Inputs=|+-
  T*m : Outport
  wires:
  Gain1/1 -> Sum1/2
  Sum1/1 -> T*m/1
  Gain2/1 -> Sum1/1
  Gain/1 -> Sum1/3
  θm*/1 -> Sum2/1
  Sum/1 -> Gain/1  "eω"
  θm/1 -> Sum2/2
  ωm*/1 -> Sum/1
  ωm/1 -> Sum/2
  Integrator1/1 -> Gain2/1  "e∫θ"
  Sum2/1 -> Gain1/1, Integrator1/1  "eθ"

== system SimulacionesDT_LUCIA_con_integral/Sistema con Controlador de Torque Equivalente y sensores ideales1/Planta (Modelo Global No Lineal) ==
  note: Sistema Global No Lineal
  Vabc : Inport  OutDataTypeStr=Bus: Vabc
  T_ld : Inport  Port=2
  g : Inport  Port=3
  T°amb : Inport  Port=4
  Id(0) : Inport  Port=5
  ~θm : Inport  Port=6
  Bus Selector : BusSelector  OutputSignals=Vd,Vq,V0
  Gain : Gain  Gain=Pp
  Subsistema Electromagnetico : Subsystem
  Subsistema Mecanico Equivalente : Subsystem
  Subsistema Termico : Subsystem
  Transformada Directa de Park : Subsystem
  Transformada Inversa de Park : Subsystem  ReferencedSubsystem=Transformada_Inversa_de_Park_I
  θm : Outport
  Iabc : Outport  Port=2  OutDataTypeStr=Bus: Iabc
  T°s : Outport  Port=3
  ωm : Outport  Port=4
  Tm : Outport  Port=5
  wires:
  Id(0)/1 -> Subsistema Electromagnetico/6(Id(0))
  Transformada Inversa de Park/1 -> Iabc/1  "Iabc"
  Bus Selector/3 -> Subsistema Electromagnetico/5(V0)  "<V0>"
  Bus Selector/2 -> Subsistema Electromagnetico/4(Vq)  "<Vq>"
  Bus Selector/1 -> Subsistema Electromagnetico/3(Vd)  "<Vd>"
  Transformada Directa de Park/1(Vdq0) -> Bus Selector/1
  g/1 -> Subsistema Mecanico Equivalente/3(g)
  T°amb/1 -> Subsistema Termico/2(T°amb)
  Vabc/1 -> Transformada Directa de Park/1(Vabc)
  T_ld/1 -> Subsistema Mecanico Equivalente/2(T_ld)
  Gain/1 -> Subsistema Electromagnetico/2(ωr)
  Subsistema Termico/1(R_s) -> Subsistema Electromagnetico/1(R_s)
  Subsistema Electromagnetico/2(T_m) -> Tm/1, Subsistema Mecanico Equivalente/1(T_m)  "Tm"
  Subsistema Mecanico Equivalente/2(θm) -> θm/1, Transformada Inversa de Park/2, Transformada Directa de Park/2(θm)  "θm"
  Subsistema Mecanico Equivalente/1(ωm) -> ωm/1, Gain/1  "ωm"
  Subsistema Electromagnetico/1(Idq0) -> Transformada Inversa de Park/1, Subsistema Termico/1(Idq0)  "Idq0"
  Subsistema Termico/2(T°s) -> T°s/1  "T°s"
  ~θm/1 -> Subsistema Mecanico Equivalente/4(~θm)

== system SimulacionesDT_LUCIA_con_integral/Sistema con Controlador de Torque Equivalente y sensores ideales1/Transformada_Directa_de_Park_I ==
  Iabc : Inport  OutDataTypeStr=Bus: Iabc
  θm : Inport  Port=2
  Ancho_abc : SignalSpecification  Dimensions=3
  Bus Creator : BusCreator  Inputs=3
  Bus to Vector : BusToVector
  Demux : Demux  Outputs=3
  Gain3 : Gain  Gain=Pp
  Park Transform : eeTransforms/Park Transform  AxisAlignment=Q-axis  PowerInvariant=off
      settings: LibrarySourceBlock=|
      | ee_sl_lib/Mathematical
      | Transforms/Park Transform
  Idq0 : Outport  OutDataTypeStr=Bus: Idq0
  wires:
  Ancho_abc/1 -> Park Transform/1
  Bus to Vector/1 -> Ancho_abc/1
  θm/1 -> Gain3/1
  Iabc/1 -> Bus to Vector/1
  Bus Creator/1 -> Idq0/1
  Demux/2 -> Bus Creator/2  "Iq"
  Demux/3 -> Bus Creator/3  "I0"
  Demux/1 -> Bus Creator/1  "Id"
  Park Transform/1 -> Demux/1  "Idq0"
  Gain3/1 -> Park Transform/2

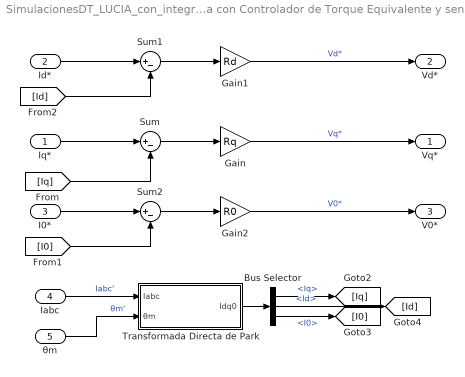
== system SimulacionesDT_LUCIA_con_integral/Sistema con Controlador de Torque Equivalente y sensores ideales/Modulador de Torque Equivalente/Lazo de Control de Corrientes Virtuales ==
  Iq* : Inport
  Id* : Inport  Port=2
  I0* : Inport  Port=3
  Iabc : Inport  Port=4
  θm : Inport  Port=5
  Bus Selector : BusSelector  OutputSignals=Iq,Id,I0
  Gain : Gain  Gain=Rq
  Gain1 : Gain  Gain=Rd
  Gain2 : Gain  Gain=R0
  Sum : Sum  Inputs=|+-
  Sum1 : Sum  Inputs=|+-
  Sum2 : Sum  Inputs=|+-
  Transformada Directa de Park : Subsystem
  Vq* : Outport
  Vd* : Outport  Port=2
  V0* : Outport  Port=3
  wires:
  Bus Selector/1 -> [Iq]  "<Iq>"
  θm/1 -> Transformada Directa de Park/2(θm)  "θm'"
  Iabc/1 -> Transformada Directa de Park/1(Iabc)  "Iabc'"
  Transformada Directa de Park/1(Idq0) -> Bus Selector/1
  Bus Selector/3 -> [I0]  "<I0>"
  Bus Selector/2 -> [Id]  "<Id>"
  I0*/1 -> Sum2/1
  [I0] -> Sum2/2
  Sum2/1 -> Gain2/1
  Gain2/1 -> V0*/1  "V0*"
  Sum/1 -> Gain/1
  [Id] -> Sum1/2
  [Iq] -> Sum/2
  Gain1/1 -> Vd*/1  "Vd*"
  Iq*/1 -> Sum/1
  Id*/1 -> Sum1/1
  Gain/1 -> Vq*/1  "Vq*"
  Sum1/1 -> Gain1/1

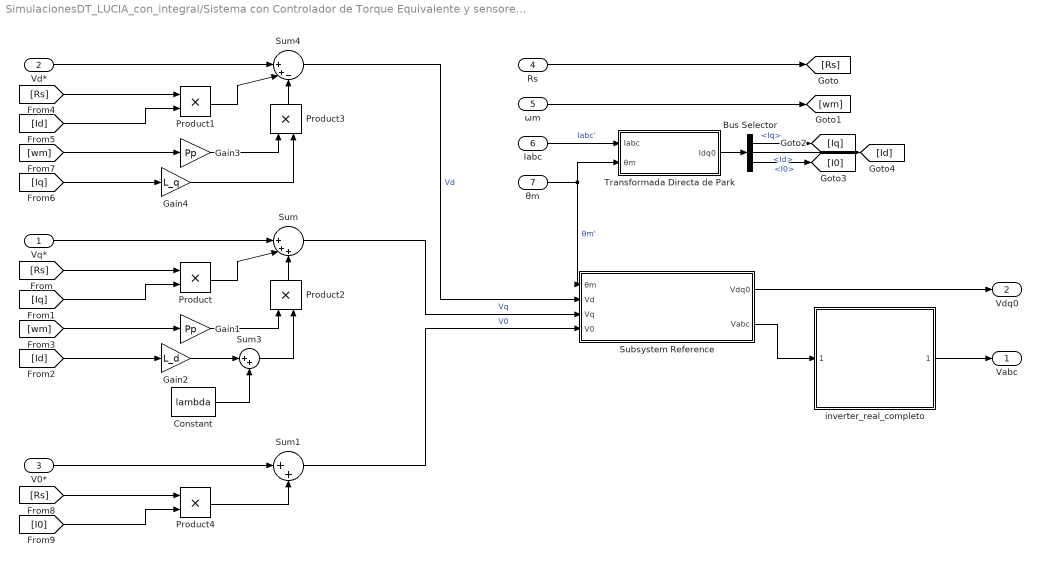
== system SimulacionesDT_LUCIA_con_integral/Sistema con Controlador de Torque Equivalente y sensores ideales/Modulador de Torque Equivalente/Modulador de Tensiones Virtuales ==
  Vq* : Inport
  Vd* : Inport  Port=2
  V0* : Inport  Port=3
  Rs : Inport  Port=4
  ωm : Inport  Port=5
  Iabc : Inport  Port=6
  θm : Inport  Port=7
  Bus Selector : BusSelector  OutputSignals=Iq,Id,I0
  Constant : Constant  Value=lambda
  Gain1 : Gain  Gain=Pp
  Gain2 : Gain  Gain=L_d
  Gain3 : Gain  Gain=Pp
  Gain4 : Gain  Gain=L_q
  Product{,1..4} (5 alike) : Product
  Subsystem Reference : Subsystem
  Sum : Sum  Inputs=||+++
  Sum1 : Sum  Inputs=|++
  Sum3 : Sum  Inputs=|++
  Sum4 : Sum  Inputs=||++-
  Transformada Directa de Park : Subsystem
  inverter_real_completo : Subsystem  ReferencedSubsystem=inverter_real_completo
  Vabc : Outport
  Vdq0 : Outport  Port=2
  wires:
  Product4/1 -> Sum1/2
  V0*/1 -> Sum1/1
  [Rs] -> Product4/1
  [I0] -> Product4/2
  [Id] -> Product1/2
  Product3/1 -> Sum4/3
  Gain4/1 -> Product3/2
  Vd*/1 -> Sum4/1
  [Rs] -> Product1/1
  Gain3/1 -> Product3/1
  [Iq] -> Gain4/1
  Product1/1 -> Sum4/2
  [wm] -> Gain3/1
  [Iq] -> Product/2
  Gain1/1 -> Product2/1
  Sum3/1 -> Product2/2
  [wm] -> Gain1/1
  Product2/1 -> Sum/3
  Gain2/1 -> Sum3/1
  [Id] -> Gain2/1
  Constant/1 -> Sum3/2
  Product/1 -> Sum/2
  [Rs] -> Product/1
  Vq*/1 -> Sum/1
  Bus Selector/2 -> [Id]  "<Id>"
  Bus Selector/3 -> [I0]  "<I0>"
  Bus Selector/1 -> [Iq]  "<Iq>"
  ωm/1 -> [wm]
  Rs/1 -> [Rs]
  Subsystem Reference/2(Vabc) -> inverter_real_completo/1
  inverter_real_completo/1 -> Vabc/1
  θm/1 -> Subsystem Reference/1(θm), Transformada Directa de Park/2(θm)  "θm'"
  Transformada Directa de Park/1(Idq0) -> Bus Selector/1
  Iabc/1 -> Transformada Directa de Park/1(Iabc)  "Iabc'"
  Subsystem Reference/1(Vdq0) -> Vdq0/1
  Sum4/1 -> Subsystem Reference/2(Vd)  "Vd"
  Sum/1 -> Subsystem Reference/3(Vq)  "Vq"
  Sum1/1 -> Subsystem Reference/4(V0)  "V0"

== system SimulacionesDT_LUCIA_con_integral/Sistema con Controlador de Torque Equivalente y sensores ideales/Modulador de Torque Equivalente/Modulador y Compensación de Torque ==
  T*m : Inport
  Iabc : Inport  Port=2
  θm : Inport  Port=3
  ωm : Inport  Port=4
  g : Inport  Port=5
  Bus Selector : BusSelector  OutputSignals=Id
  Constant : Constant  Value=lambda
  Divide : Product  Inputs=*/
  Gain1 : Gain  Gain=1/r
  Gain2 : Gain  Gain=k_l/r
  Gain3 : Gain  Gain=b_eq
  Gain4 : Gain  Gain=L_d - L_q
  Gain5 : Gain  Gain=3/2*Pp
  Product : Product
  Sin : Trigonometry
  Sum1 : Sum  Inputs=++|
  Sum2 : Sum  Inputs=|++
  Sum3 : Sum  Inputs=++|
  Transformada Directa de Park : Subsystem
  Iq* : Outport
  wires:
  Divide/1 -> Iq*/1  "Iq*"
  T*m/1 -> Sum2/1
  Iabc/1 -> Transformada Directa de Park/2(Iabc)  "Iabc'"
  θm/1 -> Gain1/1, Transformada Directa de Park/1(θm)  "θm'"
  Transformada Directa de Park/1(Idq0) -> Bus Selector/1
  Gain4/1 -> Sum1/1
  Constant/1 -> Sum1/2
  Sum1/1 -> Gain5/1
  Sum2/1 -> Divide/1
  Gain5/1 -> Divide/2
  Bus Selector/1 -> Gain4/1  "<Id>"
  Gain1/1 -> Sin/1
  Sin/1 -> Gain2/1
  Product/1 -> Sum3/2
  Gain2/1 -> Product/2
  g/1 -> Product/1  "g"
  ωm/1 -> Gain3/1  "ωm"
  Gain3/1 -> Sum3/1  "ωe"
  Sum3/1 -> Sum2/2

== system SimulacionesDT_LUCIA_con_integral/Sistema con Controlador de Torque Equivalente y sensores ideales/Modulador de Torque Equivalente/Subsystem ==
  T°s : Inport
  Constant1 : Constant  Value=T_sREF
  Constant2 : Constant
  Gain5 : Gain  Gain=alpha_Cu
  Gain6 : Gain  Gain=R_sREF
  Sum3 : Sum  Inputs=+-|
  Sum4 : Sum  Inputs=|++
  R_s : Outport
  wires:
  Sum3/1 -> Gain5/1
  Sum4/1 -> Gain6/1
  Constant2/1 -> Sum4/2
  Constant1/1 -> Sum3/2
  Gain6/1 -> R_s/1  "R_s"
  Gain5/1 -> Sum4/1
  T°s/1 -> Sum3/1

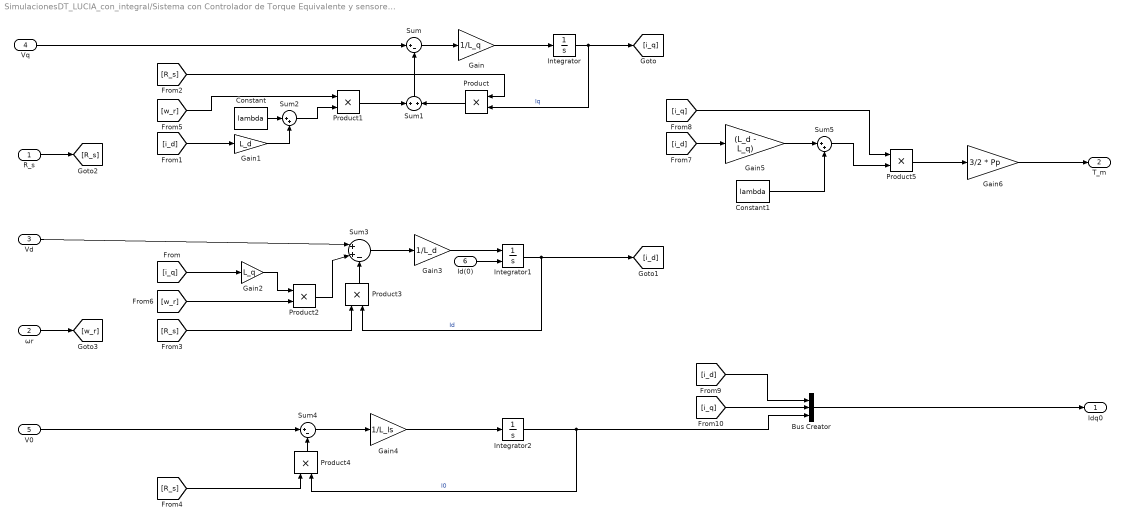
== system SimulacionesDT_LUCIA_con_integral/Sistema con Controlador de Torque Equivalente y sensores ideales/Planta (Modelo Global No Lineal)/Subsistema Electromagnetico ==
  R_s : Inport
  ωr : Inport  Port=2
  Vd : Inport  Port=3
  Vq : Inport  Port=4
  V0 : Inport  Port=5
  Id(0) : Inport  Port=6
  Bus Creator : BusCreator  Inputs=3
  Constant : Constant  Value=lambda
  Constant1 : Constant  Value=lambda
  Gain : Gain  Gain=1/L_q
  Gain1 : Gain  Gain=L_d
  Gain2 : Gain  Gain=L_q
  Gain3 : Gain  Gain=1/L_d
  Gain4 : Gain  Gain=1/L_ls
  Gain5 : Gain  Gain=(L_d - L_q)
  Gain6 : Gain  Gain=3/2 * Pp
  Integrator : Integrator  InitialCondition=init_Iq
  Integrator1 : Integrator  InitialConditionSource=external  InitialCondition=init_Id
  Integrator2 : Integrator  InitialCondition=init_I0
  Product{,1..5} (6 alike) : Product
  Sum : Sum  Inputs=|+-
  Sum1 : Sum
  Sum2 : Sum  Inputs=|++
  Sum3 : Sum  Inputs=|++-
  Sum4 : Sum  Inputs=|+-
  Sum5 : Sum  Inputs=|++
  Idq0 : Outport
  T_m : Outport  Port=2
  wires:
  [i_q] -> Bus Creator/2
  [i_d] -> Bus Creator/1
  Id(0)/1 -> Integrator1/2
  Bus Creator/1 -> Idq0/1
  [i_q] -> Product5/1
  [i_d] -> Gain5/1
  [w_r] -> Product1/1
  ωr/1 -> [w_r]
  [R_s] -> Product4/1
  [R_s] -> Product3/1
  R_s/1 -> [R_s]
  [i_d] -> Gain1/1
  Gain6/1 -> T_m/1
  Product5/1 -> Gain6/1
  Constant1/1 -> Sum5/2
  Integrator1/1 -> Product3/2, [i_d]  "Id"
  Sum5/1 -> Product5/2
  Gain5/1 -> Sum5/1
  V0/1 -> Sum4/1
  Sum4/1 -> Gain4/1
  Gain4/1 -> Integrator2/1
  Integrator2/1 -> Product4/2, Bus Creator/3  "I0"
  Product4/1 -> Sum4/2
  Vd/1 -> Sum3/1
  Sum3/1 -> Gain3/1
  Gain3/1 -> Integrator1/1
  Product3/1 -> Sum3/3
  Gain/1 -> Integrator/1
  Vq/1 -> Sum/1
  Sum/1 -> Gain/1
  Constant/1 -> Sum2/1
  Sum2/1 -> Product1/2
  Gain1/1 -> Sum2/2
  Product1/1 -> Sum1/1
  Sum1/1 -> Sum/2
  Product/1 -> Sum1/2
  [R_s] -> Product/1
  Integrator/1 -> [i_q], Product/2  "Iq"
  [i_q] -> Gain2/1
  Product2/1 -> Sum3/2
  Gain2/1 -> Product2/1
  [w_r] -> Product2/2

== system SimulacionesDT_LUCIA_con_integral/Sistema con Controlador de Torque Equivalente y sensores ideales/Planta (Modelo Global No Lineal)/Subsistema Mecanico Equivalente ==
  note: $\theta_m$
  note: $\omega_m$
  note: $\dot{\omega}_m$
  note: $T_{ld}$
  note: $T_m$
  T_m : Inport
  T_ld : Inport  Port=2
  g : Inport  Port=3
  Gain : Gain  Gain=1/r
  Gain1 : Gain  Gain=b_eq
  Gain2 : Gain  Gain=k_l/r
  Gain3 : Gain  Gain=1/J_eq
  Gain4 : Gain  Gain=1/r
  Integrator : Integrator  InitialCondition=init_w
  Integrator1 : Integrator  InitialCondition=init_theta
  Product : Product
  Sin : Trigonometry
  Sum : Sum  Inputs=|+-
  Sum1 : Sum  Inputs=+++
  ωm : Outport
  θm : Outport  Port=2
  wires:
  Integrator1/1 -> θm/1, Gain4/1
  Integrator/1 -> Gain1/1, Integrator1/1, ωm/1
  g/1 -> Product/1
  Product/1 -> Sum1/2
  T_ld/1 -> Gain/1
  Gain4/1 -> Sin/1
  Gain3/1 -> Integrator/1
  Gain1/1 -> Sum1/3
  Sin/1 -> Gain2/1
  Gain/1 -> Sum1/1
  Gain2/1 -> Product/2
  Sum1/1 -> Sum/2
  T_m/1 -> Sum/1
  Sum/1 -> Gain3/1

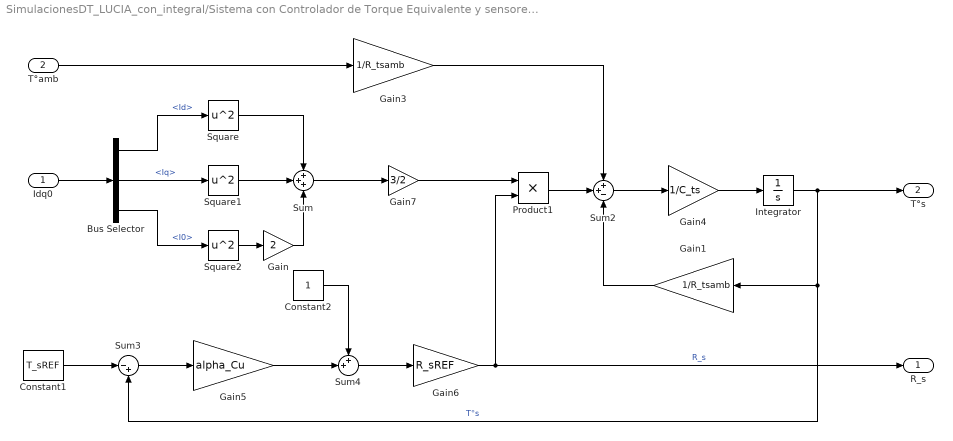
== system SimulacionesDT_LUCIA_con_integral/Sistema con Controlador de Torque Equivalente y sensores ideales/Planta (Modelo Global No Lineal)/Subsistema Termico ==
  Idq0 : Inport
  T°amb : Inport  Port=2
  Bus Selector : BusSelector  OutputSignals=Id,Iq,I0
  Constant1 : Constant  Value=T_sREF
  Constant2 : Constant
  Gain : Gain  Gain=2
  Gain1 : Gain  Gain=1/R_tsamb
  Gain3 : Gain  Gain=1/R_tsamb
  Gain4 : Gain  Gain=1/C_ts
  Gain5 : Gain  Gain=alpha_Cu
  Gain6 : Gain  Gain=R_sREF
  Gain7 : Gain  Gain=3/2
  Integrator : Integrator  InitialCondition=init_Ts
  Product1 : Product
  Square : Math  Operator=square
  Square1 : Math  Operator=square
  Square2 : Math  Operator=square
  Sum : Sum  Inputs=+++
  Sum2 : Sum  Inputs=++-
  Sum3 : Sum  Inputs=|-+
  Sum4 : Sum  Inputs=++|
  R_s : Outport
  T°s : Outport  Port=2
  wires:
  Bus Selector/3 -> Square2/1  "<I0>"
  Bus Selector/1 -> Square/1  "<Id>"
  Constant2/1 -> Sum4/1
  Idq0/1 -> Bus Selector/1
  Gain3/1 -> Sum2/1
  Gain1/1 -> Sum2/3
  Gain4/1 -> Integrator/1
  Product1/1 -> Sum2/2
  Square/1 -> Sum/1
  Sum2/1 -> Gain4/1
  Square2/1 -> Gain/1
  Sum/1 -> Gain7/1
  T°amb/1 -> Gain3/1
  Sum3/1 -> Gain5/1
  Gain5/1 -> Sum4/2
  Gain/1 -> Sum/3
  Constant1/1 -> Sum3/1
  Sum4/1 -> Gain6/1
  Gain7/1 -> Product1/1
  Gain6/1 -> Product1/2, R_s/1  "R_s"
  Integrator/1 -> T°s/1, Gain1/1, Sum3/2  "T°s"
  Square1/1 -> Sum/2
  Bus Selector/2 -> Square1/1  "<Iq>"

== system SimulacionesDT_LUCIA_con_integral/Sistema con Controlador de Torque Equivalente y sensores ideales/Planta (Modelo Global No Lineal)/Transformada Directa de Park ==
  Vabc : Inport  OutDataTypeStr=Bus: Vabc
  θm : Inport  Port=2
  Bus Creator : BusCreator  Inputs=3
  Demux : Demux  Outputs=3
  Gain3 : Gain  Gain=Pp
  MATLAB Function2 : MATLAB Function  Commented=on  TreatAsAtomicUnit=on
  Park Transform : eeTransforms/Park Transform  AxisAlignment=Q-axis  PowerInvariant=off
      settings: LibrarySourceBlock=|
      | ee_sl_lib/Mathematical
      | Transforms/Park Transform
  Vdq0 : Outport  OutDataTypeStr=Bus: Vdq0
  wires:
  Gain3/1 -> Park Transform/2
  Demux/1 -> Bus Creator/1  "Vd"
  Demux/3 -> Bus Creator/3  "V0"
  Demux/2 -> Bus Creator/2  "Vq"
  Bus Creator/1 -> Vdq0/1
  θm/1 -> Gain3/1
  Park Transform/1 -> Demux/1  "v_dq0"
  Vabc/1 -> Park Transform/1

== system SimulacionesDT_LUCIA_con_integral/Sistema con Controlador de Torque Equivalente y sensores ideales1/Modulador de Torque Equivalente/Lazo de Control de Corrientes Virtuales ==
  Iq* : Inport
  Id* : Inport  Port=2
  I0* : Inport  Port=3
  Iabc : Inport  Port=4
  θm : Inport  Port=5
  Bus Selector : BusSelector  OutputSignals=Iq,Id,I0
  Gain : Gain  Gain=Rq
  Gain1 : Gain  Gain=Rd
  Gain2 : Gain  Gain=R0
  Sum : Sum  Inputs=|+-
  Sum1 : Sum  Inputs=|+-
  Sum2 : Sum  Inputs=|+-
  Transformada Directa de Park : Subsystem
  Vq* : Outport
  Vd* : Outport  Port=2
  V0* : Outport  Port=3
  wires:
  Bus Selector/1 -> [Iq]  "<Iq>"
  θm/1 -> Transformada Directa de Park/2(θm)  "θm'"
  Iabc/1 -> Transformada Directa de Park/1(Iabc)  "Iabc'"
  Transformada Directa de Park/1(Idq0) -> Bus Selector/1
  Bus Selector/3 -> [I0]  "<I0>"
  Bus Selector/2 -> [Id]  "<Id>"
  I0*/1 -> Sum2/1
  [I0] -> Sum2/2
  Sum2/1 -> Gain2/1
  Gain2/1 -> V0*/1  "V0*"
  Sum/1 -> Gain/1
  [Id] -> Sum1/2
  [Iq] -> Sum/2
  Gain1/1 -> Vd*/1  "Vd*"
  Iq*/1 -> Sum/1
  Id*/1 -> Sum1/1
  Gain/1 -> Vq*/1  "Vq*"
  Sum1/1 -> Gain1/1

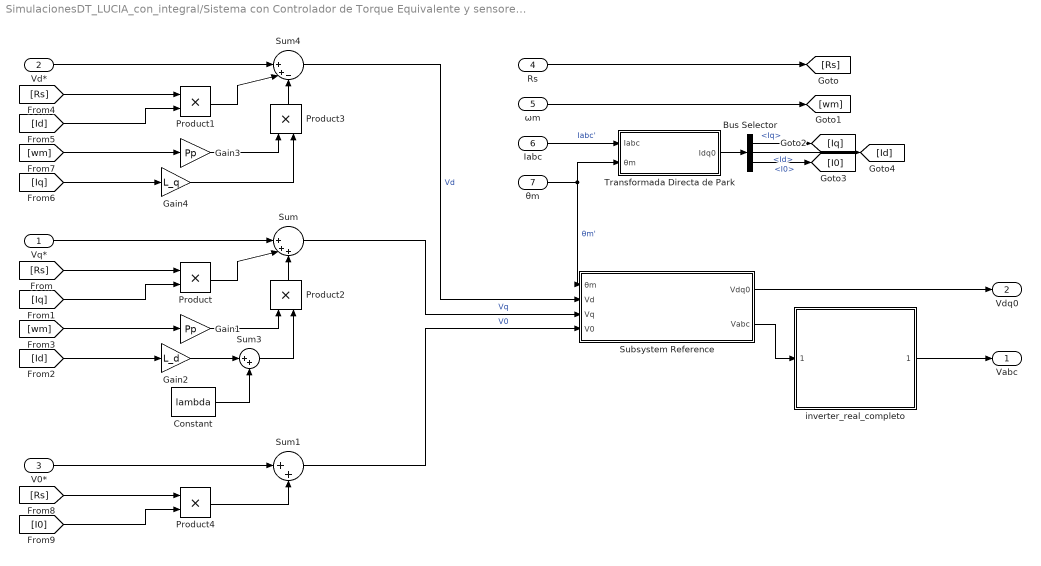
== system SimulacionesDT_LUCIA_con_integral/Sistema con Controlador de Torque Equivalente y sensores ideales1/Modulador de Torque Equivalente/Modulador de Tensiones Virtuales ==
  Vq* : Inport
  Vd* : Inport  Port=2
  V0* : Inport  Port=3
  Rs : Inport  Port=4
  ωm : Inport  Port=5
  Iabc : Inport  Port=6
  θm : Inport  Port=7
  Bus Selector : BusSelector  OutputSignals=Iq,Id,I0
  Constant : Constant  Value=lambda
  Gain1 : Gain  Gain=Pp
  Gain2 : Gain  Gain=L_d
  Gain3 : Gain  Gain=Pp
  Gain4 : Gain  Gain=L_q
  Product{,1..4} (5 alike) : Product
  Subsystem Reference : Subsystem
  Sum : Sum  Inputs=||+++
  Sum1 : Sum  Inputs=|++
  Sum3 : Sum  Inputs=|++
  Sum4 : Sum  Inputs=||++-
  Transformada Directa de Park : Subsystem
  inverter_real_completo : Subsystem  ReferencedSubsystem=inverter_real_completo
  Vabc : Outport
  Vdq0 : Outport  Port=2
  wires:
  Product4/1 -> Sum1/2
  V0*/1 -> Sum1/1
  [Rs] -> Product4/1
  [I0] -> Product4/2
  [Id] -> Product1/2
  Product3/1 -> Sum4/3
  Gain4/1 -> Product3/2
  Vd*/1 -> Sum4/1
  [Rs] -> Product1/1
  Gain3/1 -> Product3/1
  [Iq] -> Gain4/1
  Product1/1 -> Sum4/2
  [wm] -> Gain3/1
  [Iq] -> Product/2
  Gain1/1 -> Product2/1
  Sum3/1 -> Product2/2
  [wm] -> Gain1/1
  Product2/1 -> Sum/3
  Gain2/1 -> Sum3/1
  [Id] -> Gain2/1
  Constant/1 -> Sum3/2
  Product/1 -> Sum/2
  [Rs] -> Product/1
  Vq*/1 -> Sum/1
  Bus Selector/2 -> [Id]  "<Id>"
  Bus Selector/3 -> [I0]  "<I0>"
  Bus Selector/1 -> [Iq]  "<Iq>"
  ωm/1 -> [wm]
  Rs/1 -> [Rs]
  Subsystem Reference/2(Vabc) -> inverter_real_completo/1
  inverter_real_completo/1 -> Vabc/1
  θm/1 -> Subsystem Reference/1(θm), Transformada Directa de Park/2(θm)  "θm'"
  Transformada Directa de Park/1(Idq0) -> Bus Selector/1
  Iabc/1 -> Transformada Directa de Park/1(Iabc)  "Iabc'"
  Subsystem Reference/1(Vdq0) -> Vdq0/1
  Sum4/1 -> Subsystem Reference/2(Vd)  "Vd"
  Sum/1 -> Subsystem Reference/3(Vq)  "Vq"
  Sum1/1 -> Subsystem Reference/4(V0)  "V0"

== system SimulacionesDT_LUCIA_con_integral/Sistema con Controlador de Torque Equivalente y sensores ideales1/Modulador de Torque Equivalente/Modulador y Compensación de Torque ==
  T*m : Inport
  Iabc : Inport  Port=2
  θm : Inport  Port=3
  ωm : Inport  Port=4
  g : Inport  Port=5
  Bus Selector : BusSelector  OutputSignals=Id
  Constant : Constant  Value=lambda
  Divide : Product  Inputs=*/
  Gain1 : Gain  Gain=1/r
  Gain2 : Gain  Gain=k_l/r
  Gain3 : Gain  Gain=b_eq
  Gain4 : Gain  Gain=L_d - L_q
  Gain5 : Gain  Gain=3/2*Pp
  Product : Product
  Sin : Trigonometry
  Sum1 : Sum  Inputs=++|
  Sum2 : Sum  Inputs=|++
  Sum3 : Sum  Inputs=++|
  Transformada Directa de Park : Subsystem
  Iq* : Outport
  wires:
  Divide/1 -> Iq*/1  "Iq*"
  T*m/1 -> Sum2/1
  Iabc/1 -> Transformada Directa de Park/2(Iabc)  "Iabc'"
  θm/1 -> Gain1/1, Transformada Directa de Park/1(θm)  "θm'"
  Transformada Directa de Park/1(Idq0) -> Bus Selector/1
  Gain4/1 -> Sum1/1
  Constant/1 -> Sum1/2
  Sum1/1 -> Gain5/1
  Sum2/1 -> Divide/1
  Gain5/1 -> Divide/2
  Bus Selector/1 -> Gain4/1  "<Id>"
  Gain1/1 -> Sin/1
  Sin/1 -> Gain2/1
  Product/1 -> Sum3/2
  Gain2/1 -> Product/2
  g/1 -> Product/1  "g"
  ωm/1 -> Gain3/1  "ωm"
  Gain3/1 -> Sum3/1  "ωe"
  Sum3/1 -> Sum2/2
